simulink model "LAB3_CrazyFlie_2026_ros2_template"  (R2025b)
settings: Solver=ode45  StartTime=0.0  StopTime=inf  MaxStep=0.1  RelTol=1e-3  EnableMultiTasking=on
PreLoadFcn:
  | % load parameters of the default quadrotor
  | disp('Quadrotor parameters loaded by PreLoadFcn')
  | mdl_quadrotor
undefined symbols (not defined in the file): angular, linear, rot2
libraries: ros2lib x3, simulink_extras x3
settings Model: Creator=corkep  LastModifiedBy=lizar
settings SolverCC: AlgebraicLoopSolver=TrustRegion
settings DataIOCC: LimitDataPoints=on  ReturnWorkspaceOutputs=off
settings OptimizationCC: ReuseModelBlockBuffer=off  ExpressionDepthLimit=2147483647.0  LifeSpan=inf
settings DebuggingCC: UnderspecifiedInitializationDetection=Classic  MergeDetectMultiDrivingBlocksExec=none  SolverPrmCheckMsg=warning  UnconnectedInputMsg=warning  UnconnectedOutputMsg=warning  UnconnectedLineMsg=warning  AllowSymbolicDim=off  StateNameClashWarn=warning  SFUnexpectedBacktrackingDiag=warning  SFNoUnconditionalDefaultTransitionDiag=warning  SFExecutionAtInitializationDiag=none  ArithmeticOperatorsInVariantConditions=warning
settings HardwareCC: ProdBitPerPointer=32.0  ProdBitPerSizeT=32.0  ProdBitPerPtrDiffT=32.0  ProdLargestAtomicFloat=None  ProdIntDivRoundTo=Undefined  ProdEndianess=Unspecified  ProdWordSize=32.0  ProdHWDeviceType=32-bit Generic
settings ModelReferenceCC: EnableRefExpFcnMdlSchedulingChecks=on  PropagateSignalLabelsOutOfModel=off
settings SFSimCC: SimUseLocalCustomCode=off  CustomCodeUndefinedFunction=UseInterfaceOnly
settings RTWCC: RTWUseLocalCustomCode=off  GPUComputeCapability=3.5  DLArmComputeVersion=19.05
settings CodeAppCC: StateflowObjectComments=on
settings GRTTargetCC: TargetLangStandard=C89/C90 (ANSI)  CombineOutputUpdateFcns=off  GRTInterface=on
settings ConfigComp: CovMetricSettings=dw  CovSaveCumulativeToWorkspaceVar=on  CovSaveSingleToWorkspaceVar=on  CovExternalEMLEnable=off  CovSFcnEnable=off

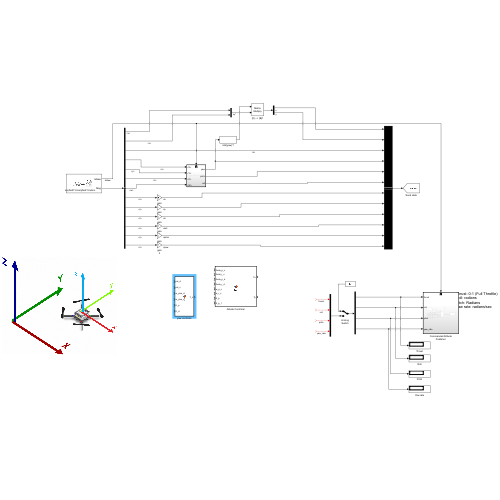
[thumbnail: Simulink's stored preview of the top-level diagram]
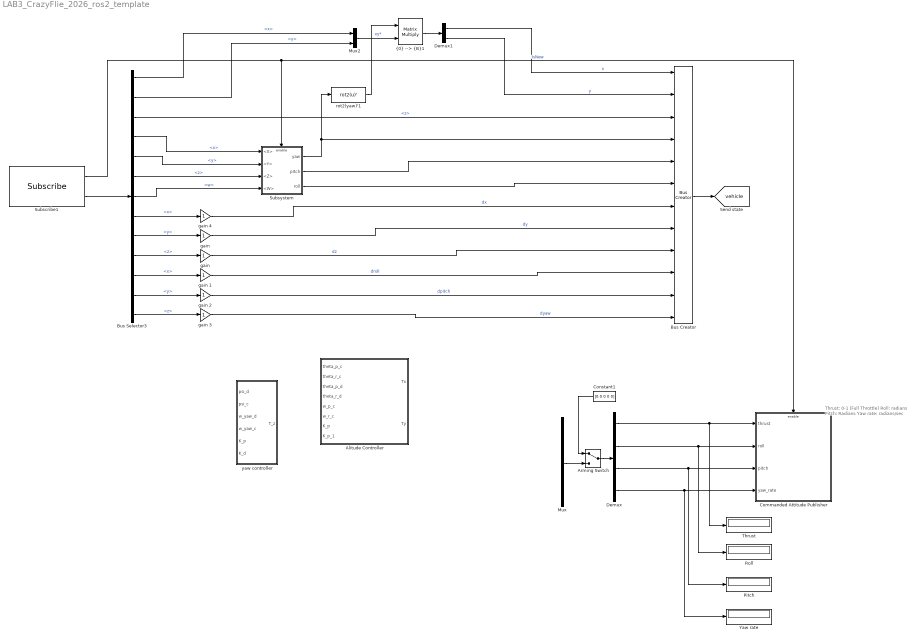
== system LAB3_CrazyFlie_2026_ros2_template ==
  note: Thrust: 0-1 (Full Throttle)
      | Roll: radians
      | Pitch: Radians
      | Yaw rate: radians/sec
  Alitude Controller : MATLAB Function  TreatAsAtomicUnit=on
  Arming Switch : ManualSwitch
  Bus Creator : BusCreator  Inputs=12
  Bus Selector3 : BusSelector  OutputSignals=pose.pose.position.x,pose.pose.position.y,pose.pose.position.z,pose.pose.orientation.x,pose.pose.orientation.y,pose.pose.orientation.z,pose.pose.orientation.w,twist.twist.linear.x,twist.twist.linear.y,twist.twist.linear.z,twist.twist.angular.x,twist.twist.angular.y,twist.twist.angular.z
  Commanded Attitude Publisher : Subsystem
  Constant1 : Constant  Value=[0.0 0 0 0]
  Demux : Demux
  Demux1 : Demux  Outputs=2
  Mux : Mux
  Mux2 : Mux  Inputs=2
  Pitch : Display
  Roll : Display
  Subscribe1 : ros2lib/Subscribe  topicSource=Select from ROS network  topic=/vicon/crazyflie211/crazyflie211/odom  messageType=nav_msgs/Odometry  sampleTime=-1  QOSHistory=Keep last  QOSDepth=1  QOSReliability=Reliable  QOSDurability=Volatile  QOSDeadline=Inf  QOSLifespan=Inf  QOSLiveliness=Automatic  QOSLeaseDuration=Inf  QOSAvoidROSNamespaceConventions=off
  Subsystem : Subsystem
  Thrust : Display
  Yaw rate : Display
  gain : Gain
  gain {,1..4} (5 alike) : Gain
  rot2(yaw)'1 : MATLABFcn  MATLABFcn=rot2(u)'  OutputDimensions=[2 2]  Output1D=off
  yaw controller : MATLAB Function  TreatAsAtomicUnit=on
  "{0} --> {B}1" : Product  Multiplication=Matrix(*)  RndMeth=Zero
  tag scope: vehicle=global
  wires:
  Bus Selector3/11 -> gain 1/1  "<x>"
  Bus Selector3/13 -> gain 3/1  "<z>"
  Bus Selector3/10 -> "gain "/1  "<z>"
  Bus Selector3/9 -> gain/1  "<y>"
  Bus Selector3/8 -> gain 4/1  "<x>"
  Bus Selector3/3 -> Bus Creator/3  "<z>"
  Bus Creator/1 -> [vehicle]
  Bus Selector3/12 -> gain 2/1  "<y>"
  Subscribe1/2 -> Bus Selector3/1
  Mux2/1 -> "{0} --> {B}1"/2  "xy*"
  "{0} --> {B}1"/1 -> Demux1/1
  Demux1/1 -> Bus Creator/1  "x"
  Demux1/2 -> Bus Creator/2  "y"
  Bus Selector3/2 -> Mux2/2  "<y>"
  rot2(yaw)'1/1 -> "{0} --> {B}1"/1
  "gain "/1 -> Bus Creator/9  "dz"
  gain 1/1 -> Bus Creator/10  "droll"
  gain 2/1 -> Bus Creator/11  "dpitch"
  gain 3/1 -> Bus Creator/12  "dyaw"
  Subsystem/1(yaw) -> rot2(yaw)'1/1, Bus Creator/4
  Bus Selector3/4 -> Subsystem/1(<X>)  "<x>"
  Bus Selector3/5 -> Subsystem/2(<Y>)  "<y>"
  Bus Selector3/6 -> Subsystem/3(<Z>)  "<z>"
  Bus Selector3/7 -> Subsystem/4(<W>)  "<w>"
  Subsystem/2(pitch) -> Bus Creator/5
  Subsystem/3(roll) -> Bus Creator/6
  Bus Selector3/1 -> Mux2/1  "<x>"
  gain 4/1 -> Bus Creator/7  "dx"
  gain/1 -> Bus Creator/8  "dy"
  Subscribe1/1 -> Subsystem/Enable, Commanded Attitude Publisher/Enable  "IsNew"
  Demux/1 -> Thrust/1, Commanded Attitude Publisher/1(thrust)
  Demux/2 -> Roll/1, Commanded Attitude Publisher/2(roll)
  Demux/3 -> Pitch/1, Commanded Attitude Publisher/3(pitch)
  Demux/4 -> Yaw rate/1, Commanded Attitude Publisher/4(yaw_rate)
  Constant1/1 -> Arming Switch/1
  Arming Switch/1 -> Demux/1
  Mux/1 -> Arming Switch/2
  ? -> Mux/1  "thrust"
  ? -> Mux/2  "roll"
  ? -> Mux/3  "pitch"
  ? -> Mux/4  "yaw_rate"

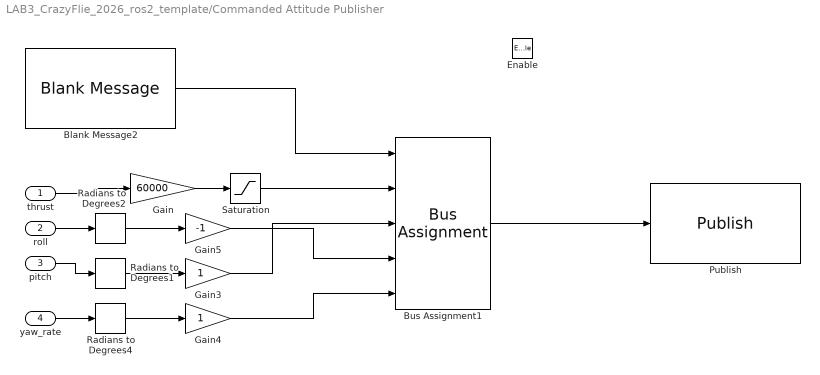
== system LAB3_CrazyFlie_2026_ros2_template/Commanded Attitude Publisher ==
  thrust : Inport
  roll : Inport  Port=2
  pitch : Inport  Port=3
  yaw_rate : Inport  Port=4
  Enable : EnablePort
  Blank Message2 : ros2lib/Blank Message  messageClass=Message  entityType=geometry_msgs/Twist  messageType=geometry_msgs/Twist  SampleTime=1/30
  Bus Assignment1 : BusAssignment  DialogController=Simulink.DDGSource_BusAssignment  AssignedSignals=linear.z,linear.x,linear.y,angular.z
  Gain : Gain  Gain=60000
  Gain3 : Gain
  Gain4 : Gain
  Gain5 : Gain  Gain=-1
  Publish : ros2lib/Publish  topicSource=Select from ROS network  topic=/cf231/cmd_vel_legacy  messageType=geometry_msgs/Twist  QOSHistory=Keep last  QOSDepth=1  QOSReliability=Reliable  QOSDurability=Volatile  QOSDeadline=Inf  QOSLifespan=Inf  QOSLiveliness=Automatic  QOSLeaseDuration=Inf  QOSAvoidROSNamespaceConventions=off
  Radians to Degrees1 : simulink_extras/Transformations/Radians to Degrees
  Radians to Degrees2 : simulink_extras/Transformations/Radians to Degrees
  Radians to Degrees4 : simulink_extras/Transformations/Radians to Degrees
  Saturation : Saturate  UpperLimit=60000  LowerLimit=0
  wires:
  Bus Assignment1/1 -> Publish/1
  Blank Message2/1 -> Bus Assignment1/1
  thrust/1 -> Gain/1
  Gain/1 -> Saturation/1
  Saturation/1 -> Bus Assignment1/2
  Gain5/1 -> Bus Assignment1/4
  Radians to Degrees2/1 -> Gain5/1
  Radians to Degrees1/1 -> Gain3/1
  Radians to Degrees4/1 -> Gain4/1
  roll/1 -> Radians to Degrees2/1
  pitch/1 -> Radians to Degrees1/1
  Gain3/1 -> Bus Assignment1/3
  yaw_rate/1 -> Radians to Degrees4/1
  Gain4/1 -> Bus Assignment1/5

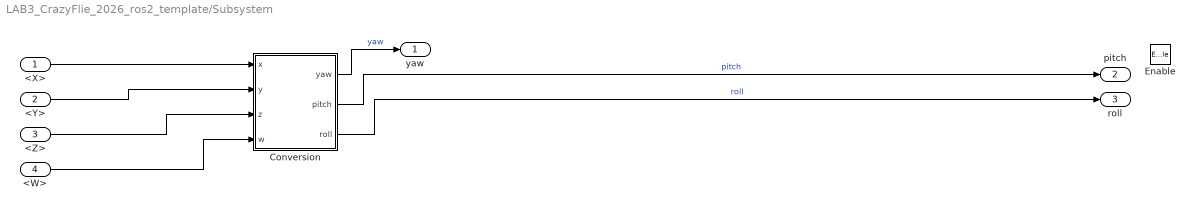
== system LAB3_CrazyFlie_2026_ros2_template/Subsystem ==
  <X> : Inport
  <Y> : Inport  Port=2
  <Z> : Inport  Port=3
  <W> : Inport  Port=4
  Enable : EnablePort
  Conversion : MATLAB Function  TreatAsAtomicUnit=on
  yaw : Outport
  pitch : Outport  Port=2
  roll : Outport  Port=3
  wires:
  Conversion/1(yaw) -> yaw/1  "yaw"
  <X>/1 -> Conversion/1(x)
  Conversion/2(pitch) -> pitch/1  "pitch"
  <W>/1 -> Conversion/4(w)
  <Y>/1 -> Conversion/2(y)
  Conversion/3(roll) -> roll/1  "roll"
  <Z>/1 -> Conversion/3(z)

== matlab function LAB3_CrazyFlie_2026_ros2_template/Subsystem/Conversion ==
  data: yaw output; x input; y input; z input; w input; pitch output; roll output
function [yaw,pitch,roll]  = quat2eul(x,y,z,w)
%#codegen

% Convert the quaternion to a yaw angle (zyx euler angle)
eul = quat2eul([w,x,y,z]);
yaw = eul(1);
roll = eul(3);
pitch = eul(2);

end

== matlab function LAB3_CrazyFlie_2026_ros2_template/Alitude Controller ==
  data: theta_p_c input; Tx output; theta_r_c input; Ty output; theta_p_d input; theta_r_d input; w_p_c input; w_r_c input; K_p input; K_p_1 input
function [Tx, Ty] = fcn(theta_p_c,theta_r_c,theta_p_d,theta_r_d,w_p_c,w_r_c,K_p,K_p_1)

w_r_d=K_p(theta_r_c-theta_r_d);
w_p_d=K_p(theta_p_c-theta_p_d);
Tx=K_p_1(w_p_d-w_p_c);
Ty=K_p_1(w_r_c-w_r_d);

== matlab function LAB3_CrazyFlie_2026_ros2_template/yaw controller ==
  data: psi_d input; T_z output; psi_c input; w_yaw_d input; w_yaw_c input; K_p input; K_d input
function T_z = fcn(psi_d,psi_c,w_yaw_d,w_yaw_c,K_p,K_d)



T_z=K_p(psi_d-psi_c)+K_d(w_yaw_d-w_yaw_c);
